simulink model "rectify"  (R2026b)
settings: Solver=VariableStepAuto
settings Model: Creator=nimnagunarathna  LastModifiedBy=nimnagunarathna

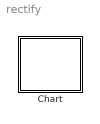
== system rectify ==
  Chart : Stateflow chart  TreatAsAtomicUnit=on

== stateflow chart rectify/Chart ==
